simulink model "s_c_nbe_m1k"  (R2016b)
settings: Solver=VariableStepAuto  StartTime=0.0  StopTime=1000  RelTol=1e-3  EnableMultiTasking=on
undefined symbols (not defined in the file): Coeffs, fft_stages, n_taps, output_bits, pfb_coeff_gen_calc, xengbits
libraries: xbsIndex_r4 x23639, casper_library_misc x65, casper_library_scopes x4, xbsReplacements_r4 x4, xps_library x3
(part 31 of 198)

== system s_c_nbe_m1k/tvg_tone_levels ==
  sim_1 : Inport
  sim_2 : Inport  Port=2
  sim_3 : Inport  Port=3
  sim_4 : Inport  Port=4
  convert1_{1..4} (4 alike) : DataTypeConversion  OutDataTypeStr=fixdt('ufix8_En7')  LockScale=on
  convert2_{1..4} (4 alike) : DataTypeConversion  OutDataTypeStr=fixdt('ufix8_En0')  ConvertRealWorld=Stored Integer (SI)  LockScale=on
  gain_1 : Gain  Gain=16777216
  gain_2 : Gain  Gain=65536
  gain_3 : Gain  Gain=256
  gain_4 : Gain
  io_delay : xbsIndex_r4/Delay  rst=off  infoeditControl=Selection of Reset will increase slice count due to use of real FFs and instead of SRLs  en=off  latency=0  reg_retiming=on  dbl_ovrd=off  block_type=delay
      settings: infoedit=Hardware notes: A delay line is a chain, each link of which is an SRL16 or SRL32 followed by a flip-flop.
  reint{1..4} (4 alike) : xbsIndex_r4/Reinterpret  force_arith_type=on  arith_type="Signed  (2's comp)"  force_bin_pt=on  bin_pt=7  block_type=reinterpret
  s_c_nbe_m1k_tvg_tone_levels_user_data_out : xbsIndex_r4/Gateway In  gui_display_data_type=Fixed-point  arith_type=Unsigned  n_bits=32  bin_pt=0  preci_type=Single  exp_width=8  frac_width=24  rows=1  columns=1  quantization="Round  (unbiased: +/- Inf)"  overflow=Saturate  period=1  UseAsADC=off  ADCChannel='1'  interface=None  automatic_assignment=on  address_offset=hex2dec('00')  intf_name=''  intf_description=''  default_value=0  timing_constraint=None  locs_specified=off  LOCs={}  io_standard={}  inherit_from_input=off  hdl_port=on  dbl_ovrd=off  block_type=gatewayin
  sim_add : Sum  Inputs=++++  OutDataTypeStr=uint32
  slice_p0i : xbsIndex_r4/Slice  nbits=8  boolean_output=off  mode=Lower Bit Location + Width  bit1=0  base1=MSB of Input  bit0=16  base0=LSB of Input  dbl_ovrd=off  block_type=slice
  slice_p0r : xbsIndex_r4/Slice  nbits=8  boolean_output=off  mode=Lower Bit Location + Width  bit1=0  base1=MSB of Input  bit0=24  base0=LSB of Input  dbl_ovrd=off  block_type=slice
  slice_p1i : xbsIndex_r4/Slice  nbits=8  boolean_output=off  mode=Lower Bit Location + Width  bit1=0  base1=MSB of Input  bit0=0  base0=LSB of Input  dbl_ovrd=off  block_type=slice
  slice_p1r : xbsIndex_r4/Slice  nbits=8  boolean_output=off  mode=Lower Bit Location + Width  bit1=0  base1=MSB of Input  bit0=8  base0=LSB of Input  dbl_ovrd=off  block_type=slice
  in_p0r : Outport
  in_p0i : Outport  Port=2
  in_p1r : Outport  Port=3
  in_p1i : Outport  Port=4
  wires:
  s_c_nbe_m1k_tvg_tone_levels_user_data_out/1 -> io_delay/1
  sim_add/1 -> s_c_nbe_m1k_tvg_tone_levels_user_data_out/1
  sim_1/1 -> convert1_1/1
  convert1_1/1 -> convert2_1/1
  convert2_1/1 -> gain_1/1
  gain_1/1 -> sim_add/1
  io_delay/1 -> slice_p0r/1, slice_p0i/1, slice_p1r/1, slice_p1i/1
  slice_p0r/1 -> reint1/1
  reint1/1 -> in_p0r/1
  sim_2/1 -> convert1_2/1
  convert1_2/1 -> convert2_2/1
  convert2_2/1 -> gain_2/1
  gain_2/1 -> sim_add/2
  slice_p0i/1 -> reint2/1
  reint2/1 -> in_p0i/1
  sim_3/1 -> convert1_3/1
  convert1_3/1 -> convert2_3/1
  convert2_3/1 -> gain_3/1
  gain_3/1 -> sim_add/3
  slice_p1r/1 -> reint3/1
  reint3/1 -> in_p1r/1
  sim_4/1 -> convert1_4/1
  convert1_4/1 -> convert2_4/1
  convert2_4/1 -> gain_4/1
  gain_4/1 -> sim_add/4
  slice_p1i/1 -> reint4/1
  reint4/1 -> in_p1i/1

== system s_c_nbe_m1k/tvg_tone_targets ==
  sim_1 : Inport
  sim_2 : Inport  Port=2
  convert1_1 : DataTypeConversion  OutDataTypeStr=fixdt('ufix11_En0')  LockScale=on
  convert1_2 : DataTypeConversion  OutDataTypeStr=fixdt('ufix11_En0')  LockScale=on
  convert2_1 : DataTypeConversion  OutDataTypeStr=fixdt('ufix11_En0')  ConvertRealWorld=Stored Integer (SI)  LockScale=on
  convert2_2 : DataTypeConversion  OutDataTypeStr=fixdt('ufix11_En0')  ConvertRealWorld=Stored Integer (SI)  LockScale=on
  gain_1 : Gain  Gain=2048
  gain_2 : Gain
  io_delay : xbsIndex_r4/Delay  rst=off  infoeditControl=Selection of Reset will increase slice count due to use of real FFs and instead of SRLs  en=off  latency=0  reg_retiming=on  dbl_ovrd=off  block_type=delay
      settings: infoedit=Hardware notes: A delay line is a chain, each link of which is an SRL16 or SRL32 followed by a flip-flop.
  reint1 : xbsIndex_r4/Reinterpret  force_arith_type=on  arith_type=Unsigned  force_bin_pt=on  bin_pt=0  block_type=reinterpret
  reint2 : xbsIndex_r4/Reinterpret  force_arith_type=on  arith_type=Unsigned  force_bin_pt=on  bin_pt=0  block_type=reinterpret
  s_c_nbe_m1k_tvg_tone_targets_user_data_out : xbsIndex_r4/Gateway In  gui_display_data_type=Fixed-point  arith_type=Unsigned  n_bits=32  bin_pt=0  preci_type=Single  exp_width=8  frac_width=24  rows=1  columns=1  quantization="Round  (unbiased: +/- Inf)"  overflow=Saturate  period=1  UseAsADC=off  ADCChannel='1'  interface=None  automatic_assignment=on  address_offset=hex2dec('00')  intf_name=''  intf_description=''  default_value=0  timing_constraint=None  locs_specified=off  LOCs={}  io_standard={}  inherit_from_input=off  hdl_port=on  dbl_ovrd=off  block_type=gatewayin
  sim_add : Sum  OutDataTypeStr=uint32
  slice_p0 : xbsIndex_r4/Slice  nbits=11  boolean_output=off  mode=Lower Bit Location + Width  bit1=0  base1=MSB of Input  bit0=11  base0=LSB of Input  dbl_ovrd=off  block_type=slice
  slice_p1 : xbsIndex_r4/Slice  nbits=11  boolean_output=off  mode=Lower Bit Location + Width  bit1=0  base1=MSB of Input  bit0=0  base0=LSB of Input  dbl_ovrd=off  block_type=slice
  in_p0 : Outport
  in_p1 : Outport  Port=2
  wires:
  s_c_nbe_m1k_tvg_tone_targets_user_data_out/1 -> io_delay/1
  sim_add/1 -> s_c_nbe_m1k_tvg_tone_targets_user_data_out/1
  sim_1/1 -> convert1_1/1
  convert1_1/1 -> convert2_1/1
  convert2_1/1 -> gain_1/1
  gain_1/1 -> sim_add/1
  io_delay/1 -> slice_p0/1, slice_p1/1
  slice_p0/1 -> reint1/1
  reint1/1 -> in_p0/1
  sim_2/1 -> convert1_2/1
  convert1_2/1 -> convert2_2/1
  convert2_2/1 -> gain_2/1
  gain_2/1 -> sim_add/2
  slice_p1/1 -> reint2/1
  reint2/1 -> in_p1/1

== system s_c_nbe_m1k/tx_metadata ==
  convert1_1 : DataTypeConversion  OutDataTypeStr=fixdt('ufix16_En0')  LockScale=on
  convert1_2 : DataTypeConversion  OutDataTypeStr=fixdt('ufix8_En0')  LockScale=on
  convert2_1 : DataTypeConversion  OutDataTypeStr=fixdt('ufix16_En0')  ConvertRealWorld=Stored Integer (SI)  LockScale=on
  convert2_2 : DataTypeConversion  OutDataTypeStr=fixdt('ufix8_En0')  ConvertRealWorld=Stored Integer (SI)  LockScale=on
  gain_1 : Gain  Gain=256
  gain_2 : Gain
  io_delay : xbsIndex_r4/Delay  rst=off  infoeditControl=Selection of Reset will increase slice count due to use of real FFs and instead of SRLs  en=off  latency=0  reg_retiming=on  dbl_ovrd=off  block_type=delay
      settings: infoedit=Hardware notes: A delay line is a chain, each link of which is an SRL16 or SRL32 followed by a flip-flop.
  reint1 : xbsIndex_r4/Reinterpret  force_arith_type=on  arith_type=Unsigned  force_bin_pt=on  bin_pt=0  block_type=reinterpret
  reint2 : xbsIndex_r4/Reinterpret  force_arith_type=on  arith_type=Unsigned  force_bin_pt=on  bin_pt=0  block_type=reinterpret
  s_c_nbe_m1k_tx_metadata_user_data_out : xbsIndex_r4/Gateway In  gui_display_data_type=Fixed-point  arith_type=Unsigned  n_bits=32  bin_pt=0  preci_type=Single  exp_width=8  frac_width=24  rows=1  columns=1  quantization="Round  (unbiased: +/- Inf)"  overflow=Saturate  period=1  UseAsADC=off  ADCChannel='1'  interface=None  automatic_assignment=on  address_offset=hex2dec('00')  intf_name=''  intf_description=''  default_value=0  timing_constraint=None  locs_specified=off  LOCs={}  io_standard={}  inherit_from_input=off  hdl_port=on  dbl_ovrd=off  block_type=gatewayin
  sim_1 : Constant  Value=0
  sim_2 : Constant  Value=0
  sim_add : Sum  OutDataTypeStr=uint32
  slice_board_id : xbsIndex_r4/Slice  nbits=8  boolean_output=off  mode=Lower Bit Location + Width  bit1=0  base1=MSB of Input  bit0=0  base0=LSB of Input  dbl_ovrd=off  block_type=slice
  slice_porttx : xbsIndex_r4/Slice  nbits=16  boolean_output=off  mode=Lower Bit Location + Width  bit1=0  base1=MSB of Input  bit0=8  base0=LSB of Input  dbl_ovrd=off  block_type=slice
  in_porttx : Outport
  in_board_id : Outport  Port=2
  wires:
  s_c_nbe_m1k_tx_metadata_user_data_out/1 -> io_delay/1
  sim_add/1 -> s_c_nbe_m1k_tx_metadata_user_data_out/1
  sim_1/1 -> convert1_1/1
  convert1_1/1 -> convert2_1/1
  convert2_1/1 -> gain_1/1
  gain_1/1 -> sim_add/1
  io_delay/1 -> slice_porttx/1, slice_board_id/1
  slice_porttx/1 -> reint1/1
  reint1/1 -> in_porttx/1
  sim_2/1 -> convert1_2/1
  convert1_2/1 -> convert2_2/1
  convert2_2/1 -> gain_2/1
  gain_2/1 -> sim_add/2
  slice_board_id/1 -> reint2/1
  reint2/1 -> in_board_id/1

== system s_c_nbe_m1k/unpack ==
  note: Put the zero-padding in the correct place in
      | the header of the incoming 40gbe digitiser
      | data.
  note: 256-bit SPEAD unpack
  note: Reorder
  note: Convert to 80-bit streams
  d256 : Inport
  dv256 : Inport  Port=2
  eof256 : Inport  Port=3
  Concat : xbsIndex_r4/Concat  num_inputs=2  dbl_ovrd=off  block_type=concat
  Constant : xbsIndex_r4/Constant  const=0  gui_display_data_type=Fixed-point  arith_type=Unsigned  n_bits=12  bin_pt=0  preci_type=Single  exp_width=8  frac_width=24  explicit_period=on  period=1  equ=P=C  opselect=C  inp2=PCIN>>17  opr=+  inp1=P  carry=CIN  dbl_ovrd=off  block_type=constant
  Delay : xbsIndex_r4/Delay  rst=off  infoeditControl=Selection of Reset will increase slice count due to use of real FFs and instead of SRLs  en=off  latency=2  reg_retiming=off  dbl_ovrd=off  block_type=delay
      settings: infoedit=Hardware notes: A delay line is a chain, each link of which is an SRL16 or SRL32 followed by a flip-flop.
  Delay1 : xbsIndex_r4/Delay  rst=off  infoeditControl=Selection of Reset will increase slice count due to use of real FFs and instead of SRLs  en=on  latency=1  reg_retiming=off  dbl_ovrd=off  block_type=delay
      settings: infoedit=Hardware notes: A delay line is a chain, each link of which is an SRL16 or SRL32 followed by a flip-flop.
  Delay{10..13} (4 alike) : xbsIndex_r4/Delay  rst=off  infoeditControl=Selection of Reset will increase slice count due to use of real FFs and instead of SRLs  en=off  latency=1  reg_retiming=off  dbl_ovrd=off  block_type=delay
      settings: infoedit=Hardware notes: A delay line is a chain, each link of which is an SRL16 or SRL32 followed by a flip-flop.
  Delay{2..9} (8 alike) : xbsIndex_r4/Delay  rst=off  infoeditControl=Selection of Reset will increase slice count due to use of real FFs and instead of SRLs  en=off  latency=1  reg_retiming=on  dbl_ovrd=off  block_type=delay
      settings: infoedit=Hardware notes: A delay line is a chain, each link of which is an SRL16 or SRL32 followed by a flip-flop.
  Inverter : xbsIndex_r4/Inverter  en=off  latency=0  dbl_ovrd=off  block_type=inv
  Inverter1 : xbsIndex_r4/Inverter  en=off  latency=0  dbl_ovrd=off  block_type=inv
  Logical : xbsIndex_r4/Logical  logical_function=AND  inputs=2  en=off  latency=2  precision=Full  arith_type=Unsigned  n_bits=16  bin_pt=0  align_bp=on  dbl_ovrd=off  block_type=logical
  Logical1 : xbsIndex_r4/Logical  logical_function=AND  inputs=4  en=off  latency=1  precision=Full  arith_type=Unsigned  n_bits=16  bin_pt=0  align_bp=on  dbl_ovrd=off  block_type=logical
  Logical2 : xbsIndex_r4/Logical  logical_function=AND  inputs=4  en=off  latency=1  precision=Full  arith_type=Unsigned  n_bits=16  bin_pt=0  align_bp=on  dbl_ovrd=off  block_type=logical
  Logical4 : xbsIndex_r4/Logical  logical_function=AND  inputs=2  en=off  latency=0  precision=Full  arith_type=Unsigned  n_bits=16  bin_pt=0  align_bp=on  dbl_ovrd=off  block_type=logical
  Logical6 : xbsIndex_r4/Logical  logical_function=AND  inputs=2  en=off  latency=0  precision=Full  arith_type=Unsigned  n_bits=16  bin_pt=0  align_bp=on  dbl_ovrd=off  block_type=logical
  Relational : xbsIndex_r4/Relational  mode=a!=b  op_type=Bool  en=off  latency=2  dbl_ovrd=off  block_type=relational
  Relational1 : xbsIndex_r4/Relational  mode=a!=b  op_type=Bool  en=off  latency=0  dbl_ovrd=off  block_type=relational
  Slice : xbsIndex_r4/Slice  nbits=2  boolean_output=off  mode=Lower Bit Location + Width  bit1=0  base1=MSB of Input  bit0=0  base0=LSB of Input  dbl_ovrd=off  block_type=slice
  Slice1 : xbsIndex_r4/Slice  nbits=1  boolean_output=on  mode=Lower Bit Location + Width  bit1=0  base1=MSB of Input  bit0=0  base0=LSB of Input  dbl_ovrd=off  block_type=slice
  Slice10 : xbsIndex_r4/Slice  nbits=1  boolean_output=on  mode=Lower Bit Location + Width  bit1=0  base1=MSB of Input  bit0=0  base0=LSB of Input  dbl_ovrd=off  block_type=slice
  Slice13 : xbsIndex_r4/Slice  nbits=1  boolean_output=on  mode=Lower Bit Location + Width  bit1=0  base1=MSB of Input  bit0=1  base0=LSB of Input  dbl_ovrd=off  block_type=slice
  Slice2 : xbsIndex_r4/Slice  nbits=36  boolean_output=off  mode=Lower Bit Location + Width  bit1=0  base1=MSB of Input  bit0=2  base0=LSB of Input  dbl_ovrd=off  block_type=slice
  Slice3 : xbsIndex_r4/Slice  nbits=12  boolean_output=off  mode=Lower Bit Location + Width  bit1=0  base1=MSB of Input  bit0=0  base0=LSB of Input  dbl_ovrd=off  block_type=slice
  Slice4 : xbsIndex_r4/Slice  nbits=1  boolean_output=on  mode=Lower Bit Location + Width  bit1=0  base1=MSB of Input  bit0=1  base0=LSB of Input  dbl_ovrd=off  block_type=slice
  Slice5 : xbsIndex_r4/Slice  nbits=16  boolean_output=off  mode=Lower Bit Location + Width  bit1=0  base1=MSB of Input  bit0=32  base0=LSB of Input  dbl_ovrd=off  block_type=slice
  Slice6 : xbsIndex_r4/Slice  nbits=1  boolean_output=on  mode=Lower Bit Location + Width  bit1=0  base1=MSB of Input  bit0=0  base0=LSB of Input  dbl_ovrd=off  block_type=slice
  Slice7 : xbsIndex_r4/Slice  nbits=1  boolean_output=off  mode=Two Bit Locations  bit1=0  base1=MSB of Input  bit0=12  base0=LSB of Input  dbl_ovrd=off  block_type=slice
  Slice8 : xbsIndex_r4/Slice  nbits=1  boolean_output=off  mode=Lower Bit Location + Width  bit1=0  base1=MSB of Input  bit0=0  base0=LSB of Input  dbl_ovrd=off  block_type=slice
  Slice9 : xbsIndex_r4/Slice  nbits=2  boolean_output=off  mode=Lower Bit Location + Width  bit1=0  base1=MSB of Input  bit0=0  base0=LSB of Input  dbl_ovrd=off  block_type=slice
  Terminator{32..34,38} (4 alike) : Terminator
  adc_clip0 : Subsystem  Tag=xps:sw_reg  AncestorBlock=xps_library/software_register  mask(swreg){io_dir=To Processor, io_delay=0, sample_period=1, names=sample_cnt, bitwidths=32, bin_pts=0, arith_types=0, sim_port=off, show_format=on}
      mask prompts: io_dir "I/O direction"; io_delay "I/O delay"; sample_period "Sample period"; names "Bitfield names [msb...lsb]"; bitwidths "Bitfield widths"; bin_pts "Bitfield binary pts"; arith_types "Bitfield types, ufix=0, fix=1, bool=2"; sim_port "Provide sim input/output?"; show_format "Print format string?"
      mask help: A 32-bit software-accessible register. Can be divided into bitfields of varying widths and types using the fields in the block mask.
      mask init:
      | swreg_init(gcb)
      settings: AttributesFormatString=1output:uf32.0 = 32 bits
      mask TypeOptions io_dir: To Processor | From Processor
      mask Callback io_dir:
      | mask_enables = get_param(gcb, 'MaskEnables');
      | mask_names = get_param(gcb, 'MaskNames');
      | if strcmp(get_param(gcb, 'io_dir'), 'To Processor'),
      |     mask_enables{ismember(mask_names, 'sample_period')} = 'off';
      | else
      |     mask_enables{ismember(mask_names, 'sample_period')} = 'on';
      | end
      | set_param(gcb, 'MaskEnables', mask_enables);
  adc_clip1 : Subsystem  Tag=xps:sw_reg  AncestorBlock=xps_library/software_register  mask(swreg){io_dir=To Processor, io_delay=0, sample_period=1, names=sample_cnt, bitwidths=32, bin_pts=0, arith_types=0, sim_port=off, show_format=on}
      mask prompts: io_dir "I/O direction"; io_delay "I/O delay"; sample_period "Sample period"; names "Bitfield names [msb...lsb]"; bitwidths "Bitfield widths"; bin_pts "Bitfield binary pts"; arith_types "Bitfield types, ufix=0, fix=1, bool=2"; sim_port "Provide sim input/output?"; show_format "Print format string?"
      mask help: A 32-bit software-accessible register. Can be divided into bitfields of varying widths and types using the fields in the block mask.
      mask init:
      | swreg_init(gcb)
      settings: AttributesFormatString=1output:uf32.0 = 32 bits
      mask TypeOptions io_dir: To Processor | From Processor
      mask Callback io_dir:
      | mask_enables = get_param(gcb, 'MaskEnables');
      | mask_names = get_param(gcb, 'MaskNames');
      | if strcmp(get_param(gcb, 'io_dir'), 'To Processor'),
      |     mask_enables{ismember(mask_names, 'sample_period')} = 'off';
      | else
      |     mask_enables{ismember(mask_names, 'sample_period')} = 'on';
      | end
      | set_param(gcb, 'MaskEnables', mask_enables);
  adc_clip_cntr0 : xbsIndex_r4/Accumulator  operation=Add  n_bits=32  overflow=Wrap  scale=1  rst=off  hasbypass=off  infoeditControl=reset for floating point data type must be asserted for a minimum of 2 cycles  en=on  latency=1  msb_inp=100  msb=100  lsb=-100  use_behavioral_HDL=on  implementation=Fabric  dbl_ovrd=off  block_type=accum
  adc_clip_cntr1 : xbsIndex_r4/Accumulator  operation=Add  n_bits=32  overflow=Wrap  scale=1  rst=off  hasbypass=off  infoeditControl=reset for floating point data type must be asserted for a minimum of 2 cycles  en=on  latency=1  msb_inp=100  msb=100  lsb=-100  use_behavioral_HDL=on  implementation=Fabric  dbl_ovrd=off  block_type=accum
  bus_create : Subsystem  AncestorBlock=casper_library_flow_control/bus_create  mask(bus_create){inputNum=2}
      mask prompts: inputNum "Number of inputs:"
      mask init:
      | bus_create_init(gcb,...
      |     'inputNum', inputNum);
  bus_expand7 : Subsystem  AncestorBlock=casper_library_flow_control/bus_expand  mask(bus_expand){mode=divisions of equal size, outputNum=2, outputWidth=256, outputBinaryPt=0, outputArithmeticType=0, show_format=on, outputToWorkspace=off, variablePrefix=out, outputToModelAsWell=on}
      mask prompts: outputNum "Number of outputs:"; outputWidth "Output width:"; outputBinaryPt "Output binary point position:"; outputArithmeticType "Output arithmetic type (ufix=0, fix=1, bool=2):"; show_format "Print format string?"; outputToWorkspace "Output to workspace?"; variablePrefix "Variable name prefix:"; outputToModelAsWell "Output to model as well?"
      mask help:
      | Expands a 'bus' made using a bus_create or Xilinx
      | concat block.
      | The input will be divided into the specified number
      | of outputs with the specified arithmetic types.
      | Divisions are made from most significant bit.
      mask init: same as s_c_nbe_m1k/bus_expand1
      settings: AttributesFormatString=2 outputs: uf256.0,uf256.0,
      mask TypeOptions mode: divisions of equal size | divisions of arbitrary size
      mask Callback mode: bus_expand_callback();
      mask Callback outputWidth: bus_expand_callback();
      mask Callback outputToWorkspace: bus_expand_callback();
  constant1 : xbsIndex_r4/Constant  const=0  gui_display_data_type=Fixed-point  arith_type=Unsigned  n_bits=3  bin_pt=0  preci_type=Single  exp_width=8  frac_width=24  explicit_period=on  period=1  equ=P=C  opselect=C  inp2=PCIN>>17  opr=+  inp1=P  carry=CIN  dbl_ovrd=off  block_type=constant
  latched_time : xbsIndex_r4/Register  init=0  rst=off  en=on  dbl_ovrd=off  block_type=register
  pack_256_80 : Subsystem  mask{mux_latency=7}
      mask prompts: mux_latency "Mux latency"
      mask init:
      | annotation = sprintf('latency=%i', mux_latency);
      | set_param(gcb, 'AttributesFormatString', annotation);
      settings: AttributesFormatString=latency=7
  pad_and_barrel_shift : Subsystem
  pkt_reorder : Subsystem  mask{window_bits=5, window_size_words=160, n_bits_din=256, n_bits_flag=2, n_bits_timestamp=48 - 12}
      mask prompts: window_bits "Number of Windows to Buffer (2^?)"; window_size_words "Window size (words)"; n_bits_din "Data bit width in"; n_bits_flag "Flag bit width in"; n_bits_timestamp "Timestamp bit width"
      mask init:
      | win_nbits = ceil(log2(window_size_words));
      | fmtstr = sprintf('Buffer space: 2^%i words', window_bits + win_nbits);
      | set_param(gcb, 'AttributesFormatString', fmtstr);
      settings: AttributesFormatString=Buffer space: 2^13 words
  time48_regen : xbsIndex_r4/Concat  num_inputs=3  dbl_ovrd=off  block_type=concat
  time_pkt_cnt : xbsIndex_r4/Counter  cnt_type=Free Running  cnt_to=1  operation=Up  start_count=0  cnt_by_val=1  arith_type=Unsigned  n_bits=12-3  bin_pt=0  load_pin=off  rst=on  en=on  explicit_period=on  period=1  use_behavioral_HDL=off  implementation=Fabric  dbl_ovrd=off  block_type=counter
  unpack_feng : Subsystem  Tag=casper:spead_unpack  AncestorBlock=casper_library_communications/spead_unpack  mask(spead_unpack_mask){max_pkt_len_bits=10, header_ids=0x1600, 0x4101, 0x4103, header_ind_ids=0x4300, spead_msw=64, spead_lsw=48, spead_version=4, combine_errors=on}
      mask prompts: max_pkt_len_bits "Max pkt length, 2^? 64-bit words"; header_ids "SPEAD direct header IDs (decimal)"; header_ind_ids "SPEAD indirect address IDs (decimal)"; spead_msw "SPEAD Flavour (MSw)"; spead_lsw "SPEAD Flavour (LSw)"; spead_version "SPEAD version"; combine_errors "Combine error flags"
      mask help: This block receives a 64-bit-word stream that contains a SPEAD stream. It checks the SPEAD headers are being correctly received. It presents the user with all headers on the first valid cycle of data along with a flag to indicate a header or packet-length error.
      mask init:
      | %spead_unpack_init(gcb)
  d160 : Outport
  dv : Outport  Port=2
  time : Outport  Port=3
  recvd : Outport  Port=4
  spead_timestamp : Outport  Port=5
  tag scope: upg_barrel_dv=global, upg_barrel_eof=global, upg_barrel_hdr_edit=global, upg_of80_p0=global, upg_of80_p1=global, upg_reo_disc=global, upg_reo_dv=global, upg_reo_not_recv=global, upg_reo_recv=global, upg_reo_relock=global, upg_reo_time=global, upg_sp_0x3101=global, upg_sp_dv=global, upg_sp_eof=global, upg_sp_heapid=global, upg_sp_timestamp=global, upg_sperr_hdr=global, upg_sperr_len=global, upg_sperr_magic=global, upg_sperr_pad=global, upg_sperr_time=global
  wires:
  d256/1 -> pad_and_barrel_shift/1(data)
  pad_and_barrel_shift/1(data_out) -> [proc_d256]
  eof256/1 -> pad_and_barrel_shift/3(eof)
  pad_and_barrel_shift/2(dv_out) -> [upg_barrel_dv], [proc_dv]
  pad_and_barrel_shift/3(eof_out) -> [upg_barrel_eof], [proc_eof]
  dv256/1 -> pad_and_barrel_shift/2(dv)
  [proc_d256] -> unpack_feng/1(pkt_data)
  [proc_dv] -> unpack_feng/2(pkt_valid)
  [proc_eof] -> unpack_feng/3(pkt_eof)
  unpack_feng/1(pkt_start) -> [spead_pktstart]  "pkt_start"
  unpack_feng/2(data256) -> [spead_d256]  "d256"
  unpack_feng/3(valid256) -> [spead_dv]  "dv"
  unpack_feng/4(eof256) -> [spead_eof]  "eof"
  unpack_feng/5(magic_error) -> [spead_err_magic]  "err_magic"
  unpack_feng/6(hdr_error) -> [spead_err_hdr]  "err_hdr"
  unpack_feng/7(pad_error) -> [spead_err_pad]  "err_pad"
  unpack_feng/8(pkt_len_err) -> [spead_err_len]  "err_len"
  unpack_feng/9(hdr_heap_id) -> [spead_heapid]  "heap_id"
  unpack_feng/10(hdr_heap_size) -> Terminator32/1  "heap_size"
  unpack_feng/11(hdr_heap_offset) -> Terminator33/1  "heap_offset"
  unpack_feng/12(hdr_pkt_len) -> Terminator34/1  "pkt_len"
  unpack_feng/13(hdr5_0x1600_DIR) -> [spead_timestamp]  "timestamp"
  unpack_feng/14(hdr6_0x3101_DIR) -> [spead_0x3101]  "0x3101"
  unpack_feng/15(hdr7_0x3102_DIR) -> [spead_0x3102]  "0x3102"
  unpack_feng/16(hdr8_0x3300) -> Terminator38/1  "0x3300"
  [spead_d256] -> pkt_reorder/1(din)
  [spead_timestamp] -> Slice7/1  "spead_time"
  Slice7/1 -> pkt_reorder/2(time_in)
  [spead_0x3101] -> Slice8/1
  Slice8/1 -> pkt_reorder/3(src_in)
  [spead_eof] -> pkt_reorder/6(eof)
  [spead_dv] -> pkt_reorder/5(valid_in)
  [spead_0x3102] -> Slice9/1
  Slice9/1 -> pkt_reorder/4(flag_in)
  pkt_reorder/1(data_out) -> [reo_data]
  pkt_reorder/2(flag_out) -> [reo_flag]
  pkt_reorder/3(valid_out) -> [reo_dv]
  pkt_reorder/4(rcvd) -> [reo_recv]
  pkt_reorder/5(time_out) -> [reo_time]
  pkt_reorder/6(mcnt_relock) -> [reo_relock]
  pkt_reorder/7(discarding) -> [reo_disc]
  [reo_data] -> bus_expand7/1(bus_in)
  pad_and_barrel_shift/4(hdr_splice) -> [upg_barrel_hdr_edit]
  [reo_disc] -> [upg_reo_disc]
  [reo_relock] -> [upg_reo_relock]
  [reo_dv] -> [upg_reo_dv]
  [reo_time] -> [upg_reo_time]
  [reo_recv] -> [upg_reo_recv]
  bus_create/1(bus_out) -> Delay4/1
  pack_256_80/1(valid80) -> Delay7/1
  bus_expand7/1(msb_out2) -> pack_256_80/1(data256_p0)
  bus_expand7/2(lsb_out1) -> pack_256_80/2(data256_p1)
  [reo_dv] -> pack_256_80/3(valid)  "reo_dv"
  pack_256_80/2(data80_p0) -> bus_create/1(in1)
  pack_256_80/3(data80_p1) -> bus_create/2(in2)
  Concat/1 -> pack_256_80/4(timei)
  [reo_time] -> Concat/1
  [reo_recv] -> Concat/2
  Slice/1 -> Delay5/1
  [spead_0x3101] -> [upg_sp_0x3101]
  [spead_err_hdr] -> [upg_sperr_hdr]
  [spead_err_magic] -> [upg_sperr_magic]
  [spead_err_pad] -> [upg_sperr_pad]
  [spead_err_len] -> [upg_sperr_len]
  [spead_eof] -> [upg_sp_eof]
  [spead_dv] -> [upg_sp_dv]
  [spead_timestamp] -> [upg_sp_timestamp]
  [spead_heapid] -> [upg_sp_heapid]
  [spead_timestamp] -> Slice3/1
  Slice3/1 -> Relational/2
  Constant/1 -> Relational/1
  Relational/1 -> Logical/2
  [spead_dv] -> Delay/1
  Delay/1 -> Logical/1
  Logical/1 -> [upg_sperr_time]
  [reo_recv] -> Slice13/1, Slice6/1
  Slice6/1 -> Logical4/1
  Slice13/1 -> Logical4/2
  Logical4/1 -> Inverter/1
  Inverter/1 -> Logical6/1
  Logical6/1 -> [upg_reo_not_recv]
  [reo_dv] -> Logical6/2
  [spead_timestamp] -> Delay1/1
  [spead_dv] -> Delay1/2
  Delay1/1 -> spead_timestamp/1
  pack_256_80/5(timeo) -> Slice2/1, Slice/1
  time_pkt_cnt/1 -> time48_regen/2
  Slice2/1 -> Delay3/1, Relational1/2, Delay2/1
  constant1/1 -> time48_regen/3
  Delay2/1 -> Relational1/1
  Relational1/1 -> time_pkt_cnt/1
  Delay3/1 -> time48_regen/1
  Delay7/1 -> time_pkt_cnt/2, latched_time/2, Delay6/1
  Delay4/1 -> Delay8/1
  Delay5/1 -> Delay9/1
  pack_256_80/4(overflow) -> [upg_of80_p1], [upg_of80_p0]
  Delay6/1 -> dv/1
  Delay8/1 -> d160/1
  Delay9/1 -> recvd/1
  latched_time/1 -> time/1
  time48_regen/1 -> latched_time/1
  [spead_0x3102] -> Slice4/1, Slice5/1, Slice1/1
  Slice1/1 -> [nd_firing]
  Slice4/1 -> [adc_clip]
  Slice5/1 -> [adc_clip_cnt]
  [spead_eof] -> Logical1/1
  [adc_clip] -> Logical1/2
  [spead_dv] -> Logical1/3
  Logical1/1 -> adc_clip_cntr0/2
  [adc_clip_cnt] -> Delay10/1
  Delay10/1 -> adc_clip_cntr0/1
  [spead_0x3101] -> Slice10/1
  Slice10/1 -> [src_pol]
  [src_pol] -> Inverter1/1
  [spead_eof] -> Logical2/1
  [adc_clip] -> Logical2/2
  [spead_dv] -> Logical2/3
  Logical2/1 -> adc_clip_cntr1/2
  [adc_clip_cnt] -> Delay11/1
  Delay11/1 -> adc_clip_cntr1/1
  [src_pol] -> Logical2/4
  Inverter1/1 -> Logical1/4
  adc_clip_cntr1/1 -> Delay13/1
  adc_clip_cntr0/1 -> Delay12/1
  Delay12/1 -> adc_clip0/1(out_sample_cnt)
  Delay13/1 -> adc_clip1/1(out_sample_cnt)

== system s_c_nbe_m1k/unpack_status ==
  out_magic_err_cnt : Inport
  out_header_err_cnt : Inport  Port=2
  out_pad_err_cnt : Inport  Port=3
  out_pkt_len_err_cnt : Inport  Port=4
  out_time_err_cnt : Inport  Port=5
  assert_header_err_cnt : xbsIndex_r4/Assert  assert_type=on  type_source=Explicitly  gui_display_data_type=Fixed-point  arith_type=Unsigned  n_bits=6  bin_pt=0  preci_type=Single  exp_width=8  frac_width=24  assert_rate=off  rate_source=Explicitly  period=1  output_port=on  block_type=assert
  assert_magic_err_cnt : xbsIndex_r4/Assert  assert_type=on  type_source=Explicitly  gui_display_data_type=Fixed-point  arith_type=Unsigned  n_bits=6  bin_pt=0  preci_type=Single  exp_width=8  frac_width=24  assert_rate=off  rate_source=Explicitly  period=1  output_port=on  block_type=assert
  assert_pad_err_cnt : xbsIndex_r4/Assert  assert_type=on  type_source=Explicitly  gui_display_data_type=Fixed-point  arith_type=Unsigned  n_bits=6  bin_pt=0  preci_type=Single  exp_width=8  frac_width=24  assert_rate=off  rate_source=Explicitly  period=1  output_port=on  block_type=assert
  assert_pkt_len_err_cnt : xbsIndex_r4/Assert  assert_type=on  type_source=Explicitly  gui_display_data_type=Fixed-point  arith_type=Unsigned  n_bits=6  bin_pt=0  preci_type=Single  exp_width=8  frac_width=24  assert_rate=off  rate_source=Explicitly  period=1  output_port=on  block_type=assert
  assert_time_err_cnt : xbsIndex_r4/Assert  assert_type=on  type_source=Explicitly  gui_display_data_type=Fixed-point  arith_type=Unsigned  n_bits=6  bin_pt=0  preci_type=Single  exp_width=8  frac_width=24  assert_rate=off  rate_source=Explicitly  period=1  output_port=on  block_type=assert
  cast_gw : xbsIndex_r4/Convert  gui_display_data_type=Fixed-point  arith_type=Unsigned  n_bits=32  bin_pt=0  float_type=Single  exp_bits=8  fraction_bits=24  quantization=Truncate  overflow=Wrap  en=off  latency=1  pipeline=off  dbl_ovrd=off  block_type=convert
  concatenate : xbsIndex_r4/Concat  num_inputs=5  dbl_ovrd=off  block_type=concat
  io_delay : xbsIndex_r4/Delay  rst=off  infoeditControl=Selection of Reset will increase slice count due to use of real FFs and instead of SRLs  en=off  latency=0  reg_retiming=on  dbl_ovrd=off  block_type=delay
      settings: infoedit=Hardware notes: A delay line is a chain, each link of which is an SRL16 or SRL32 followed by a flip-flop.
  reint{1..5} (5 alike) : xbsIndex_r4/Reinterpret  force_arith_type=on  arith_type=Unsigned  force_bin_pt=on  bin_pt=0  block_type=reinterpret
  s_c_nbe_m1k_unpack_status_user_data_in : xbsIndex_r4/Gateway Out  inherit_from_input=off  hdl_port=on  rows=1  columns=1  UseAsDAC=off  DACChannel='1'  interface=None  automatic_assignment=on  address_offset=hex2dec('00')  intf_name=''  intf_description=''  timing_constraint=None  locs_specified=off  LOCs={}  io_standard={}  block_type=gatewayout
  sim_out : Terminator
  wires:
  concatenate/1 -> io_delay/1
  io_delay/1 -> cast_gw/1
  cast_gw/1 -> s_c_nbe_m1k_unpack_status_user_data_in/1
  s_c_nbe_m1k_unpack_status_user_data_in/1 -> sim_out/1
  out_magic_err_cnt/1 -> assert_magic_err_cnt/1
  assert_magic_err_cnt/1 -> reint1/1
  reint1/1 -> concatenate/1
  out_header_err_cnt/1 -> assert_header_err_cnt/1
  assert_header_err_cnt/1 -> reint2/1
  reint2/1 -> concatenate/2
  out_pad_err_cnt/1 -> assert_pad_err_cnt/1
  assert_pad_err_cnt/1 -> reint3/1
  reint3/1 -> concatenate/3
  out_pkt_len_err_cnt/1 -> assert_pkt_len_err_cnt/1
  assert_pkt_len_err_cnt/1 -> reint4/1
  reint4/1 -> concatenate/4
  out_time_err_cnt/1 -> assert_time_err_cnt/1
  assert_time_err_cnt/1 -> reint5/1
  reint5/1 -> concatenate/5

== system s_c_nbe_m1k/unpack_status1 ==
  out_pkt_cnt : Inport
  assert_pkt_cnt : xbsIndex_r4/Assert  assert_type=on  type_source=Explicitly  gui_display_data_type=Fixed-point  arith_type=Unsigned  n_bits=32  bin_pt=0  preci_type=Single  exp_width=8  frac_width=24  assert_rate=off  rate_source=Explicitly  period=1  output_port=on  block_type=assert
  cast_gw : xbsIndex_r4/Convert  gui_display_data_type=Fixed-point  arith_type=Unsigned  n_bits=32  bin_pt=0  float_type=Single  exp_bits=8  fraction_bits=24  quantization=Truncate  overflow=Wrap  en=off  latency=1  pipeline=off  dbl_ovrd=off  block_type=convert
  io_delay : xbsIndex_r4/Delay  rst=off  infoeditControl=Selection of Reset will increase slice count due to use of real FFs and instead of SRLs  en=off  latency=0  reg_retiming=on  dbl_ovrd=off  block_type=delay
      settings: infoedit=Hardware notes: A delay line is a chain, each link of which is an SRL16 or SRL32 followed by a flip-flop.
  reint1 : xbsIndex_r4/Reinterpret  force_arith_type=on  arith_type=Unsigned  force_bin_pt=on  bin_pt=0  block_type=reinterpret
  s_c_nbe_m1k_unpack_status1_user_data_in : xbsIndex_r4/Gateway Out  inherit_from_input=off  hdl_port=on  rows=1  columns=1  UseAsDAC=off  DACChannel='1'  interface=None  automatic_assignment=on  address_offset=hex2dec('00')  intf_name=''  intf_description=''  timing_constraint=None  locs_specified=off  LOCs={}  io_standard={}  block_type=gatewayout
  sim_out : Terminator
  wires:
  io_delay/1 -> cast_gw/1
  cast_gw/1 -> s_c_nbe_m1k_unpack_status1_user_data_in/1
  s_c_nbe_m1k_unpack_status1_user_data_in/1 -> sim_out/1
  out_pkt_cnt/1 -> assert_pkt_cnt/1
  assert_pkt_cnt/1 -> reint1/1
  reint1/1 -> io_delay/1

== system s_c_nbe_m1k/wb_prog_delay ==
  sync : Inport
  delay_val : Inport  Port=2
  din : Inport  Port=3
  en : Inport  Port=4
  load_val : Inport  Port=5
  Concat : xbsIndex_r4/Concat  num_inputs=2  dbl_ovrd=off  block_type=concat
  Concat1 : xbsIndex_r4/Concat  num_inputs=8  dbl_ovrd=off  block_type=concat
  Delay6 : xbsIndex_r4/Delay  rst=off  infoeditControl=Selection of Reset will increase slice count due to use of real FFs and instead of SRLs  en=off  latency=1  reg_retiming=off  dbl_ovrd=off  block_type=delay
  Slice : xbsIndex_r4/Slice  nbits=4  boolean_output=off  mode=Lower Bit Location + Width  bit1=0  base1=MSB of Input  bit0=0  base0=LSB of Input  dbl_ovrd=off  block_type=slice
  Slice2 : xbsIndex_r4/Slice  nbits=1  boolean_output=on  mode=Lower Bit Location + Width  bit1=0  base1=MSB of Input  bit0=0  base0=LSB of Input  dbl_ovrd=off  block_type=slice
  Slice3 : xbsIndex_r4/Slice  nbits=4  boolean_output=off  mode=Upper Bit Location + Width  bit1=0  base1=MSB of Input  bit0=0  base0=LSB of Input  dbl_ovrd=off  block_type=slice
  Terminator : Terminator
  Terminator1 : Terminator
  Terminator2 : Terminator
  bus_expand : Subsystem  AncestorBlock=casper_library_flow_control/bus_expand  mask(bus_expand){mode=divisions of equal size, outputNum=8, outputWidth=10, outputBinaryPt=0, outputArithmeticType=0, show_format=off, outputToWorkspace=off, variablePrefix=out, outputToModelAsWell=on}
      mask prompts: outputNum "Number of outputs:"; outputWidth "Output width:"; outputBinaryPt "Output binary point position:"; outputArithmeticType "Output arithmetic type (ufix=0, fix=1, bool=2):"; show_format "Print format string?"; outputToWorkspace "Output to workspace?"; variablePrefix "Variable name prefix:"; outputToModelAsWell "Output to model as well?"
      mask help:
      | Expands a 'bus' made using a bus_create or Xilinx
      | concat block.
      | The input will be divided into the specified number
      | of outputs with the specified arithmetic types.
      | Divisions are made from most significant bit.
      mask init: same as s_c_nbe_m1k/bus_expand1
      settings: AttributesFormatString=8 outputs
      mask TypeOptions mode: divisions of equal size | divisions of arbitrary size
      mask Callback mode: bus_expand_callback();
      mask Callback outputWidth: bus_expand_callback();
      mask Callback outputToWorkspace: bus_expand_callback();
  bus_expand1 : Subsystem  AncestorBlock=casper_library_flow_control/bus_expand  mask(bus_expand){mode=divisions of arbitrary size, outputNum=1, outputWidth=[64 64 16 16], outputBinaryPt=[32 32 15 15], outputArithmeticType=[1 1 1 1], show_format=off, outputToWorkspace=off, variablePrefix=out, outputToModelAsWell=on}
      mask prompts: outputNum "Number of outputs:"; outputWidth "Output width [msb ... lsb]:"; outputBinaryPt "Output binary point position [msb ... lsb]:"; outputArithmeticType "Output arithmetic type (ufix=0, fix=1, bool=2) [msb ... lsb]:"; show_format "Print format string?"; outputToWorkspace "Output to workspace?"; variablePrefix "Variable name prefix:"; outputToModelAsWell "Output to model as well?"
      mask help:
      | Expands a 'bus' made using a bus_create or Xilinx
      | concat block.
      | The input will be divided into the specified number
      | of outputs with the specified arithmetic types.
      | Divisions are made from most significant bit.
      mask init: same as s_c_nbe_m1k/bus_expand1
      settings: AttributesFormatString=4 outputs
      mask TypeOptions mode: divisions of equal size | divisions of arbitrary size
      mask Callback mode: bus_expand_callback();
      mask Callback outputWidth: bus_expand_callback();
      mask Callback outputToWorkspace: bus_expand_callback();
  delay_gen : Subsystem  mask{n_bits_fft_words=n_bits_fft-3, n_bits_streams=3, n_bits_fft=n_bits_fft-1, n_bits_data=10, n_bits_cd=n_bits_cd}
      mask prompts: n_bits_fft_words "FFT size (2^? data words)"; n_bits_streams "parallel data streams (2^?)"; n_bits_fft "effective FFT size (2^? bins)"; n_bits_data "data bit width"; n_bits_cd "max coarse delay (2^?)"
  delay_wideband_prog : Subsystem  AncestorBlock=casper_library_delays/delay_wideband_prog  mask(delay_wideband_prog){max_delay=16, n_inputs_bits=3, bram_latency=3, bram_type=Dual Port, async=on}
      mask prompts: max_delay "Max Delay (Sample Clks)"; n_inputs_bits "Number of Simultaneous Inputs(2^?)"; bram_latency "BRAM Latency"; bram_type "Select type of BRAM"; async "asynchronous operation"
      mask init:
      | delay_wideband_prog_init(gcb,...
      |     'max_delay',max_delay,...
      |     'n_inputs_bits',n_inputs_bits,...
      |     'bram_latency',bram_latency,...
      |     'bram_type',bram_type, ...
      |     'async', async);
      mask TypeOptions bram_type: Single Port | Dual Port
  sync_out : Outport
  data_out : Outport  Port=2
  dvalid : Outport  Port=3
  wires:
  delay_wideband_prog/4(data_out2) -> Concat1/3  "d6"
  bus_expand/1(msb_out8) -> delay_wideband_prog/4(data_in0)  "dw_in_1"
  delay_wideband_prog/2(data_out0) -> Concat1/1  "d8"
  bus_expand/4(out5) -> delay_wideband_prog/7(data_in3)  "dw_in_4"
  delay_wideband_prog/9(data_out7) -> Concat1/8  "d1"
  delay_wideband_prog/7(data_out5) -> Concat1/6  "d3"
  delay_wideband_prog/1(sync_out) -> sync_out/1
  Slice3/1 -> delay_wideband_prog/2(delay)  "delay_bs"
  bus_expand/2(out7) -> delay_wideband_prog/5(data_in1)  "dw_in_2"
  delay_wideband_prog/3(data_out1) -> Concat1/2  "d7"
  delay_wideband_prog/5(data_out3) -> Concat1/4  "d5"
  bus_expand/6(out3) -> delay_wideband_prog/9(data_in5)  "dw_in_6"
  bus_expand/7(out2) -> delay_wideband_prog/10(data_in6)  "dw_in_7"
  Slice2/1 -> delay_wideband_prog/3(ld_delay)  "ld_delay"
  delay_wideband_prog/8(data_out6) -> Concat1/7  "d2"
  delay_wideband_prog/10(dvalid) -> dvalid/1
  delay_wideband_prog/6(data_out4) -> Concat1/5  "d4"
  Concat1/1 -> data_out/1
  bus_expand/8(lsb_out1) -> delay_wideband_prog/11(data_in7)  "dw_in_8"
  bus_expand/5(out4) -> delay_wideband_prog/8(data_in4)  "dw_in_5"
  bus_expand/3(out6) -> delay_wideband_prog/6(data_in2)  "dw_in_3"
  bus_expand1/1(msb_out4) -> delay_gen/4(delay)
  bus_expand1/2(out3) -> delay_gen/5(d/dt_delay)
  bus_expand1/3(out2) -> delay_gen/6(phase)
  bus_expand1/4(lsb_out1) -> delay_gen/7(d/dt_phase)
  sync/1 -> delay_gen/1(sync_in)
  din/1 -> delay_gen/2(din)
  en/1 -> delay_gen/3(en)
  delay_val/1 -> bus_expand1/1(bus_in)
  load_val/1 -> delay_gen/8(ld)
  delay_gen/7(coarse_delay) -> Slice/1  "delay_tp"
  delay_gen/8(new_value) -> Delay6/1
  Slice/1 -> Concat/1  "delay_tp1"
  delay_gen/1(sync_out) -> [bs_sync], delay_wideband_prog/1(sync)
  Delay6/1 -> Concat/2
  delay_gen/2(dout) -> [bs_in], bus_expand/1(bus_in)
  Concat/1 -> Slice3/1, Slice2/1
  delay_gen/6(slope) -> Terminator/1
  delay_gen/5(initial_phase) -> Terminator1/1
  delay_gen/3(idx_out) -> Terminator2/1
  delay_gen/4(dvalid) -> [bs_en], delay_wideband_prog/12(en)

== system s_c_nbe_m1k/wb_prog_delay1 ==
  sync : Inport
  delay_val : Inport  Port=2
  din : Inport  Port=3
  en : Inport  Port=4
  load_val : Inport  Port=5
  Concat : xbsIndex_r4/Concat  num_inputs=2  dbl_ovrd=off  block_type=concat
  Concat1 : xbsIndex_r4/Concat  num_inputs=8  dbl_ovrd=off  block_type=concat
  Delay6 : xbsIndex_r4/Delay  rst=off  infoeditControl=Selection of Reset will increase slice count due to use of real FFs and instead of SRLs  en=off  latency=1  reg_retiming=off  dbl_ovrd=off  block_type=delay
  Slice : xbsIndex_r4/Slice  nbits=4  boolean_output=off  mode=Lower Bit Location + Width  bit1=0  base1=MSB of Input  bit0=0  base0=LSB of Input  dbl_ovrd=off  block_type=slice
  Slice2 : xbsIndex_r4/Slice  nbits=1  boolean_output=on  mode=Lower Bit Location + Width  bit1=0  base1=MSB of Input  bit0=0  base0=LSB of Input  dbl_ovrd=off  block_type=slice
  Slice3 : xbsIndex_r4/Slice  nbits=4  boolean_output=off  mode=Upper Bit Location + Width  bit1=0  base1=MSB of Input  bit0=0  base0=LSB of Input  dbl_ovrd=off  block_type=slice
  Terminator : Terminator
  Terminator1 : Terminator
  Terminator2 : Terminator
  bus_expand : Subsystem  AncestorBlock=casper_library_flow_control/bus_expand  mask(bus_expand){mode=divisions of equal size, outputNum=8, outputWidth=10, outputBinaryPt=0, outputArithmeticType=0, show_format=off, outputToWorkspace=off, variablePrefix=out, outputToModelAsWell=on}
      mask prompts: outputNum "Number of outputs:"; outputWidth "Output width:"; outputBinaryPt "Output binary point position:"; outputArithmeticType "Output arithmetic type (ufix=0, fix=1, bool=2):"; show_format "Print format string?"; outputToWorkspace "Output to workspace?"; variablePrefix "Variable name prefix:"; outputToModelAsWell "Output to model as well?"
      mask help:
      | Expands a 'bus' made using a bus_create or Xilinx
      | concat block.
      | The input will be divided into the specified number
      | of outputs with the specified arithmetic types.
      | Divisions are made from most significant bit.
      mask init: same as s_c_nbe_m1k/bus_expand1
      settings: AttributesFormatString=8 outputs
      mask TypeOptions mode: divisions of equal size | divisions of arbitrary size
      mask Callback mode: bus_expand_callback();
      mask Callback outputWidth: bus_expand_callback();
      mask Callback outputToWorkspace: bus_expand_callback();
  bus_expand1 : Subsystem  AncestorBlock=casper_library_flow_control/bus_expand  mask(bus_expand){mode=divisions of arbitrary size, outputNum=1, outputWidth=[64 64 16 16], outputBinaryPt=[32 32 15 15], outputArithmeticType=[1 1 1 1], show_format=off, outputToWorkspace=off, variablePrefix=out, outputToModelAsWell=on}
      mask prompts: outputNum "Number of outputs:"; outputWidth "Output width [msb ... lsb]:"; outputBinaryPt "Output binary point position [msb ... lsb]:"; outputArithmeticType "Output arithmetic type (ufix=0, fix=1, bool=2) [msb ... lsb]:"; show_format "Print format string?"; outputToWorkspace "Output to workspace?"; variablePrefix "Variable name prefix:"; outputToModelAsWell "Output to model as well?"
      mask help:
      | Expands a 'bus' made using a bus_create or Xilinx
      | concat block.
      | The input will be divided into the specified number
      | of outputs with the specified arithmetic types.
      | Divisions are made from most significant bit.
      mask init: same as s_c_nbe_m1k/bus_expand1
      settings: AttributesFormatString=4 outputs
      mask TypeOptions mode: divisions of equal size | divisions of arbitrary size
      mask Callback mode: bus_expand_callback();
      mask Callback outputWidth: bus_expand_callback();
      mask Callback outputToWorkspace: bus_expand_callback();
  delay_gen : Subsystem  mask{n_bits_fft_words=n_bits_fft-3, n_bits_streams=3, n_bits_fft=n_bits_fft-1, n_bits_data=10, n_bits_cd=n_bits_cd}
      mask prompts: n_bits_fft_words "FFT size (2^? data words)"; n_bits_streams "parallel data streams (2^?)"; n_bits_fft "effective FFT size (2^? bins)"; n_bits_data "data bit width"; n_bits_cd "max coarse delay (2^?)"
  delay_wideband_prog : Subsystem  AncestorBlock=casper_library_delays/delay_wideband_prog  mask(delay_wideband_prog){max_delay=16, n_inputs_bits=3, bram_latency=3, bram_type=Dual Port, async=on}
      mask prompts: max_delay "Max Delay (Sample Clks)"; n_inputs_bits "Number of Simultaneous Inputs(2^?)"; bram_latency "BRAM Latency"; bram_type "Select type of BRAM"; async "asynchronous operation"
      mask init:
      | delay_wideband_prog_init(gcb,...
      |     'max_delay',max_delay,...
      |     'n_inputs_bits',n_inputs_bits,...
      |     'bram_latency',bram_latency,...
      |     'bram_type',bram_type, ...
      |     'async', async);
      mask TypeOptions bram_type: Single Port | Dual Port
  sync_out : Outport
  data_out : Outport  Port=2
  dvalid : Outport  Port=3
  wires:
  delay_gen/4(dvalid) -> delay_wideband_prog/12(en), [bs_en]
  delay_gen/3(idx_out) -> Terminator2/1
  delay_gen/5(initial_phase) -> Terminator1/1
  delay_gen/6(slope) -> Terminator/1
  Concat/1 -> Slice2/1, Slice3/1
  delay_gen/2(dout) -> bus_expand/1(bus_in), [bs_in]
  Delay6/1 -> Concat/2
  delay_gen/1(sync_out) -> delay_wideband_prog/1(sync), [bs_sync]
  Slice/1 -> Concat/1  "delay_tp1"
  delay_gen/8(new_value) -> Delay6/1
  delay_gen/7(coarse_delay) -> Slice/1  "delay_tp"
  load_val/1 -> delay_gen/8(ld)
  delay_val/1 -> bus_expand1/1(bus_in)
  en/1 -> delay_gen/3(en)
  din/1 -> delay_gen/2(din)
  sync/1 -> delay_gen/1(sync_in)
  bus_expand1/4(lsb_out1) -> delay_gen/7(d/dt_phase)
  bus_expand1/3(out2) -> delay_gen/6(phase)
  bus_expand1/2(out3) -> delay_gen/5(d/dt_delay)
  bus_expand1/1(msb_out4) -> delay_gen/4(delay)
  bus_expand/3(out6) -> delay_wideband_prog/6(data_in2)  "dw_in_3"
  bus_expand/5(out4) -> delay_wideband_prog/8(data_in4)  "dw_in_5"
  bus_expand/8(lsb_out1) -> delay_wideband_prog/11(data_in7)  "dw_in_8"
  Concat1/1 -> data_out/1
  delay_wideband_prog/6(data_out4) -> Concat1/5  "d4"
  delay_wideband_prog/10(dvalid) -> dvalid/1
  delay_wideband_prog/8(data_out6) -> Concat1/7  "d2"
  Slice2/1 -> delay_wideband_prog/3(ld_delay)  "ld_delay"
  bus_expand/7(out2) -> delay_wideband_prog/10(data_in6)  "dw_in_7"
  bus_expand/6(out3) -> delay_wideband_prog/9(data_in5)  "dw_in_6"
  delay_wideband_prog/5(data_out3) -> Concat1/4  "d5"
  delay_wideband_prog/3(data_out1) -> Concat1/2  "d7"
  bus_expand/2(out7) -> delay_wideband_prog/5(data_in1)  "dw_in_2"
  Slice3/1 -> delay_wideband_prog/2(delay)  "delay_bs"
  delay_wideband_prog/1(sync_out) -> sync_out/1
  delay_wideband_prog/7(data_out5) -> Concat1/6  "d3"
  delay_wideband_prog/9(data_out7) -> Concat1/8  "d1"
  bus_expand/4(out5) -> delay_wideband_prog/7(data_in3)  "dw_in_4"
  delay_wideband_prog/2(data_out0) -> Concat1/1  "d8"
  bus_expand/1(msb_out8) -> delay_wideband_prog/4(data_in0)  "dw_in_1"
  delay_wideband_prog/4(data_out2) -> Concat1/3  "d6"

== system s_c_nbe_m1k/we_delay1 ==
  d : Inport
  Register0 : xbsIndex_r4/Register  init=0  rst=off  en=off  dbl_ovrd=off  block_type=register
      settings: block_version=11.4
  Register1 : xbsIndex_r4/Register  init=0  rst=off  en=off  dbl_ovrd=off  block_type=register
  q : Outport
  wires:
  Register1/1 -> q/1
  d/1 -> Register0/1
  Register0/1 -> Register1/1

== system s_c_nbe_m1k/we_delay112 ==
  d : Inport
  Register0 : xbsIndex_r4/Register  init=0  rst=off  en=off  dbl_ovrd=off  block_type=register
      settings: block_version=11.4
  Register1 : xbsIndex_r4/Register  init=0  rst=off  en=off  dbl_ovrd=off  block_type=register
  q : Outport
  wires:
  Register1/1 -> q/1
  d/1 -> Register0/1
  Register0/1 -> Register1/1

== system s_c_nbe_m1k/we_delay113 ==
  d : Inport
  Register0 : xbsIndex_r4/Register  init=0  rst=off  en=off  dbl_ovrd=off  block_type=register
      settings: block_version=11.4
  Register1 : xbsIndex_r4/Register  init=0  rst=off  en=off  dbl_ovrd=off  block_type=register
  q : Outport
  wires:
  Register0/1 -> Register1/1
  d/1 -> Register0/1
  Register1/1 -> q/1

== system s_c_nbe_m1k/we_delay114 ==
  d : Inport
  Register0 : xbsIndex_r4/Register  init=0  rst=off  en=off  dbl_ovrd=off  block_type=register
      settings: block_version=11.4
  Register1 : xbsIndex_r4/Register  init=0  rst=off  en=off  dbl_ovrd=off  block_type=register
  q : Outport
  wires:
  Register1/1 -> q/1
  d/1 -> Register0/1
  Register0/1 -> Register1/1

== system s_c_nbe_m1k/we_delay115 ==
  d : Inport
  Register0 : xbsIndex_r4/Register  init=0  rst=off  en=off  dbl_ovrd=off  block_type=register
      settings: block_version=11.4
  Register1 : xbsIndex_r4/Register  init=0  rst=off  en=off  dbl_ovrd=off  block_type=register
  q : Outport
  wires:
  Register1/1 -> q/1
  d/1 -> Register0/1
  Register0/1 -> Register1/1

== system s_c_nbe_m1k/we_delay116 ==
  d : Inport
  Register0 : xbsIndex_r4/Register  init=0  rst=off  en=off  dbl_ovrd=off  block_type=register
      settings: block_version=11.4
  Register1 : xbsIndex_r4/Register  init=0  rst=off  en=off  dbl_ovrd=off  block_type=register
  q : Outport
  wires:
  Register1/1 -> q/1
  d/1 -> Register0/1
  Register0/1 -> Register1/1

== system s_c_nbe_m1k/we_delay117 ==
  d : Inport
  Register0 : xbsIndex_r4/Register  init=0  rst=off  en=off  dbl_ovrd=off  block_type=register
      settings: block_version=11.4
  Register1 : xbsIndex_r4/Register  init=0  rst=off  en=off  dbl_ovrd=off  block_type=register
  q : Outport
  wires:
  Register0/1 -> Register1/1
  d/1 -> Register0/1
  Register1/1 -> q/1

== system s_c_nbe_m1k/we_delay124 ==
  d : Inport
  Register0 : xbsIndex_r4/Register  init=0  rst=off  en=off  dbl_ovrd=off  block_type=register
      settings: block_version=11.4
  Register1 : xbsIndex_r4/Register  init=0  rst=off  en=off  dbl_ovrd=off  block_type=register
  q : Outport
  wires:
  Register0/1 -> Register1/1
  d/1 -> Register0/1
  Register1/1 -> q/1

== system s_c_nbe_m1k/we_delay126 ==
  d : Inport
  Register0 : xbsIndex_r4/Register  init=0  rst=off  en=off  dbl_ovrd=off  block_type=register
      settings: block_version=11.4
  Register1 : xbsIndex_r4/Register  init=0  rst=off  en=off  dbl_ovrd=off  block_type=register
  q : Outport
  wires:
  Register1/1 -> q/1
  d/1 -> Register0/1
  Register0/1 -> Register1/1
